simulink model "QC_PilotTraining"  (R2026b)
settings: Solver=ode4  StopTime=inf  FixedStep=3e-4  MaxStep=1e-2  MinStep=1e-3  RelTol=1e-2  AbsTol=1e-4
libraries: sl3dlib x1
settings Model: Creator=dani  LastModifiedBy=Dani
settings SolverCC: AutoScaleAbsTol=off  EnableFixedStepZeroCrossing=on  ShapePreserveControl=EnableAll  ZeroCrossAlgorithm=Adaptive
settings DataIOCC: DSMLogging=off  ReturnWorkspaceOutputs=off  SaveOutput=off  SaveTime=off  SignalLogging=off
settings DebuggingCC: InheritedTsInSrcMsg=none
settings HardwareCC: ProdHWDeviceType=Intel->x86-64 (Linux 64)  ProdLongLongMode=on
settings RTWCC: Description=Simulink Desktop Real-Time  GPUComputeCapability=5.0  RTWCompilerOptimization=on  SystemTargetFile=sldrt.tlc  TemplateMakefile=sldrt.tmf
settings SimulinkDesktopRealTimeCC: ParMdlRefBuildCompliant=on  RealTimeExecution=kernel  TargetLibSuffix=_sldrt.a  TargetPreCompLibLocation=C:\Program Files\MATLAB\R2026b\toolbox\sldrt\lib\win64
settings SimscapeCC: SimscapeUseEnergyAccounting=on
settings ExplorerConfigSet: InternalSimMechanicsExplorerSettings=|
  | <ExplorerConfiguration>
  | 
  |   <canonicalview>default</canonicalview>
  | 
  |   <TilePanel>
  |     <TileInfo>
  |       <Tiles Columns="2" Count="2" Height="825" Rows="1" Width="1462">
  |         <Row Weight="1"/>
  |         <Column Weight="0.511665"/>
  |         <Column Weight="0.488335"/>
  |         <Tile Height="1" Width="1" X="0" Y="0"/>
  |         <Tile Height="1" Width="1" X="1" Y="0"/>
  |       </Tiles>
  |     </TileInfo>
  |     <SceneInfo>
  |       <SceneViewer>
  |         <IsThisViewStd>
  |           <IsStandardView>off</IsStandardView>
  |           <StandardViewName>Front</StandardViewName>
  |         </IsThisViewStd>
  |         <BGColor>
  |           <R>1</R>
  |           <G>1</G>
  |           <B>1</B>
  |           <A>1</A>
  |         </BGColor>
  |         <Camera>
  |           <DoPerspective>off</DoPerspective>
  |           <Position>
  |             <X>-8.7352421661405089</X>
  |             <Y>0</Y>
  |             <Z>0.34578637035021559</Z>
  |           </Position>
  |           <Center>
  |             <X>0</X>
  |             <Y>0</Y>
  |             <Z>0.34578637035021559</Z>
  |           </Center>
  |           <Up>
  |             <X>0</X>
  |             <Y>0</Y>
  |             <Z>1</Z>
  |           </Up>
  |           <XLim>1.03</XLim>
  |           <YLim>1.03</YLim>
  |           <ViewLimDist>0.01</ViewLimDist>
  |         </Camera>
  |       </SceneViewer>
  |       <SceneViewer>
  |         <IsThisViewStd>
  |           <IsStandardView>off</IsStandardView>
  |           <StandardViewName>Front</StandardViewName>
  |         </IsThisViewStd>
  |         <BGColor>
  |           <R>1</R>
  |           <G>1</G>
  |           <B>1</B>
  |           <A>1</A>
  |         </BGColor>
  |         <Camera>
  |           <DoPerspective>on</DoPerspective>
  |           <Position>
  |             <X>7.6704062163307576</X>
  |             <Y>-1.1602462844035919</Y>
  |             <Z>2</Z>
  |           </Position>
  |           <Center>
  |             <X>7.6704062163307576</X>
  |             <Y>-1.1602462844035919</Y>
  |             <Z>0</Z>
  |           </Center>
  |           <Up>
  |             <X>-0.54646337970634273</X>
  |             <Y>0.83748299961248263</Y>
  |             <Z>0</Z>
  |           </Up>
  |           <XLim>0.93261531630999717</XLim>
  |           <YLim>0.93261531630999717</YLim>
  |           <ViewLimDist>0.01</ViewLimDist>
  |         </Camera>
  |       </SceneViewer>
  |     </SceneInfo>
  |   </TilePanel>
  | 
  |   <MechEditorPanel>
  |     <GfxPanelCameraMap>
  |       <MapElement CameraMLId="Camera1" GfxPanelIndex="1"/>
  |     </GfxPanelCameraMap>
  |     <Cameras>
  |       <Camera>
  |         <Id>Camera1</Id>
  |         <Value>
  |           <Name>Camera1</Name>
  |           <NativeCamera>
  |             <PositionTrackingFeature>Camera.Camera_Frame_Pos.R</PositionTrackingFeature>
  |             <CenterTrackingFeature>Camera.Camera_Frame_target.R</CenterTrackingFeature>
  |             <UpVectorTrackingFeature>Camera.Camera_Frame_Pos.R</UpVectorTrackingFeature>
  |             <CenterTrackingOrigin>on</CenterTrackingOrigin>
  |             <UpVectorTrackingDirection>+X</UpVectorTrackingDirection>
  |           </NativeCamera>
  |         </Value>
  |       </Camera>
  |     </Cameras>
  |     <VideoCreator>
  |       <IncludeTiles>All</IncludeTiles>
  |       <IncludeTime>on</IncludeTime>
  |       <IncludeWorldFrame>off</IncludeWorldFrame>
  |       <PlaybackSpeedRatio>1</PlaybackSpeedRatio>
  |       <FrameRate>30</FrameRate>
  |       <FrameSize>auto</FrameSize>
  |       <VideoFormat>UncompressedAVI</VideoFormat>
  |     </VideoCreator>
  |   </MechEditorPanel>
  | 
  |   <PlaybackSettings>
  |     <PlaybackSpeedFactor>4</PlaybackSpeedFactor>
  |   </PlaybackSettings>
  | 
  | </ExplorerConfiguration>

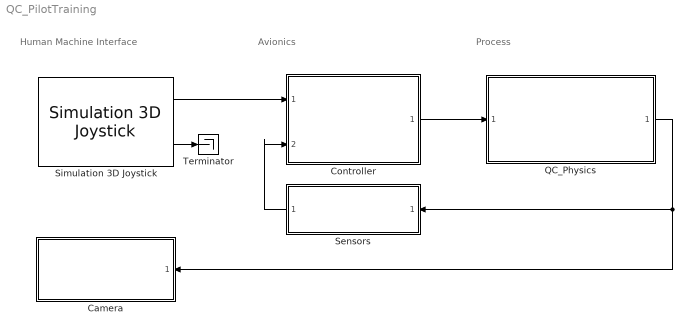
== system QC_PilotTraining ==
  note: Process
  note: Avionics
  note: Human Machine Interface
  Camera : Subsystem  ReferencedSubsystem=Camera_ViewPoint
  Controller : Subsystem  TreatAsAtomicUnit=on  SystemSampleTime=3e-4*4  ReferencedSubsystem=Controller
  QC_Physics : Subsystem  ReferencedSubsystem=QC_Physics
  Sensors : Subsystem  ReferencedSubsystem=Sensors
  Simulation 3D Joystick : sl3dlib/Simulation 3D/Hardware Interface/Simulation 3D Joystick  joyid=0  adjustports=off  forcefeed=off
  Terminator : Terminator
  wires:
  Simulation 3D Joystick/1 -> Controller/1
  Controller/1 -> QC_Physics/1
  QC_Physics/1 -> Camera/1, Sensors/1
  Sensors/1 -> Controller/2
  Simulation 3D Joystick/2 -> Terminator/1
